simulink model "Crazyflie_Sim_CrazyDreive"  (R2026b)
settings: Solver=ode15s  StopTime=20  RelTol=1e-5
InitFcn:
  | Crazyflie_Param
values from neighbouring files (symbols this model uses):
  g = 9.80665    [Crazyflie_Param.m]
  invMix = inv(Mix)    [Crazyflie_Param.m]
  Ix_drone = 2.934e-5    (= 2.934e-05)    [Crazyflie_Param.m]
  Iy_drone = 4.981e-5    (= 4.981e-05)    [Crazyflie_Param.m]
  Iz_drone = 7.646e-5    (= 7.646e-05)    [Crazyflie_Param.m]
  J = 1/12*m*(0.051^2+0.005^2)    (= 7.878e-08)    [Crazyflie_Param.m]
  K = lqr(A, B_v, Q, R)    [Crazyflie_Param.m]
  kq = 0.006    [Crazyflie_Param.m]
  l1 = 4.445    [Crazyflie_Param.m]
  m = 0.00036    [Crazyflie_Param.m]
  m_drone = 0.04316    [Crazyflie_Param.m]
  T_e = m_tot*g/4    (= 0.1093441475)    [Crazyflie_Param.m]
undefined symbols (not defined in the file or in its folder): sigbuilder_block, X, Y, Z
libraries: sm_lib x57, nesl_utility x21, slpidlib x19, fl_lib x9
(part 1 of 4)
settings Model: Creator=BKIM  LastModifiedBy=lapsi
settings DataIOCC: ReturnWorkspaceOutputs=off
settings DebuggingCC: ArithmeticOperatorsInVariantConditions=warning
settings SFSimCC: CustomCodeUndefinedFunction=UseInterfaceOnly  SimUseLocalCustomCode=off
settings RTWCC: RTWUseLocalCustomCode=off
settings CodeAppCC: StateflowObjectComments=on
settings SimscapeCC: SimscapeNormalizeSystem=off  SimscapeUseEnergyAccounting=off
settings DiagnosticsConfigSet: SimMechanicsRigidlyBoundBlock=warning

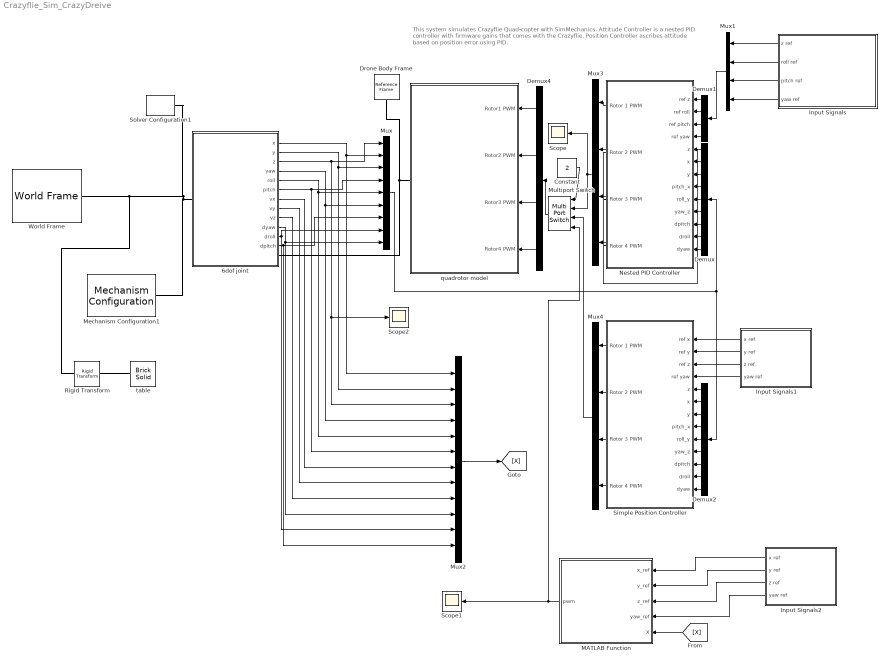
== system Crazyflie_Sim_CrazyDreive ==
  note: This system simulates Crazyflie Quad-copter with SimMechanics.
      | Attitude Controller is a nested PID controller with firmware gains that comes with the Crazyflie.
      | Position Controller ascribes attitude based on position error using PID.
  6dof joint : Subsystem
  Constant : Constant  Value=2
  Demux : Demux  Outputs=9
  Demux1 : Demux
  Demux2 : Demux  Outputs=9
  Demux4 : Demux
  Drone Body Frame : sm_lib/Frames and Transforms/Reference Frame
  Input Signals : Subsystem  Tag=STV Subsys  LoadFcn=sigbuilder_block('load');  StartFcn=sigbuilder_block('start');  StopFcn=sigbuilder_block('stop');  ClipboardFcn=sigbuilder_block('clipboard');  mask(Sigbuilder block){tuvar=[0:10]}
      mask help: Simulink:masks:SigbuilderBlock_MD
      mask init:
      | if ~strcmp(get_param(bdroot(gcbh),'SimulationStatus'),'stopped') tuvar = sigbuilder_block('maskInit'); end
      settings: CopyFcn=sigbuilder_block('copy');  DeleteFcn=sigbuilder_block('delete');  ModelCloseFcn=sigbuilder_block('modelClose');  PreSaveFcn=sigbuilder_block('preSave');  PauseFcn=sigbuilder_block('pause');  ContinueFcn=sigbuilder_block('continue');  NameChangeFcn=sigbuilder_block('namechange');  OpenFcn=sigbuilder_block('open',[6 0 1428 756 ]);  CloseFcn=sigbuilder_block('close');
      mask Display: plot(0, 0, 100, 100,[2, 2, 32, 32, 2], [68, 8, 8, 68, 68],[32, 2], [38, 38], [32, 19, 2],[53, 60, 44], [32, 17, 17, 2],[16, 16, 31, 31]);txt = getActiveGroup(gcbh);text(2, 100, txt,'verticalAlignment', 'top');
  Input Signals1 : Subsystem  Tag=STV Subsys  LoadFcn=sigbuilder_block('load');  StartFcn=sigbuilder_block('start');  StopFcn=sigbuilder_block('stop');  ClipboardFcn=sigbuilder_block('clipboard');  mask(Sigbuilder block){tuvar=[0:10]}
      mask help: Simulink:masks:SigbuilderBlock_MD
      mask init:
      | if ~strcmp(get_param(bdroot(gcbh),'SimulationStatus'),'stopped') tuvar = sigbuilder_block('maskInit'); end
      settings: CopyFcn=sigbuilder_block('copy');  DeleteFcn=sigbuilder_block('delete');  ModelCloseFcn=sigbuilder_block('modelClose');  PreSaveFcn=sigbuilder_block('preSave');  PauseFcn=sigbuilder_block('pause');  ContinueFcn=sigbuilder_block('continue');  NameChangeFcn=sigbuilder_block('namechange');  OpenFcn=sigbuilder_block('open',[441.75 141 756 505.5 ]);  CloseFcn=sigbuilder_block('close');
      mask Display: plot(0, 0, 100, 100,[2, 2, 32, 32, 2], [68, 8, 8, 68, 68],[32, 2], [38, 38], [32, 19, 2],[53, 60, 44], [32, 17, 17, 2],[16, 16, 31, 31]);txt = getActiveGroup(gcbh);text(2, 100, txt,'verticalAlignment', 'top');
  Input Signals2 : Subsystem  Tag=STV Subsys  LoadFcn=sigbuilder_block('load');  StartFcn=sigbuilder_block('start');  StopFcn=sigbuilder_block('stop');  ClipboardFcn=sigbuilder_block('clipboard');  mask(Sigbuilder block){tuvar=[0:10]}
      mask help: Simulink:masks:SigbuilderBlock_MD
      mask init:
      | if ~strcmp(get_param(bdroot(gcbh),'SimulationStatus'),'stopped') tuvar = sigbuilder_block('maskInit'); end
      settings: CopyFcn=sigbuilder_block('copy');  DeleteFcn=sigbuilder_block('delete');  ModelCloseFcn=sigbuilder_block('modelClose');  PreSaveFcn=sigbuilder_block('preSave');  PauseFcn=sigbuilder_block('pause');  ContinueFcn=sigbuilder_block('continue');  NameChangeFcn=sigbuilder_block('namechange');  OpenFcn=sigbuilder_block('open',[441.75 141 756 505.5 ]);  CloseFcn=sigbuilder_block('close');
      mask Display: plot(0, 0, 100, 100,[2, 2, 32, 32, 2], [68, 8, 8, 68, 68],[32, 2], [38, 38], [32, 19, 2],[53, 60, 44], [32, 17, 17, 2],[16, 16, 31, 31]);txt = getActiveGroup(gcbh);text(2, 100, txt,'verticalAlignment', 'top');
  MATLAB Function : MATLAB Function  TreatAsAtomicUnit=on
  Mechanism Configuration1 : sm_lib/Utilities/Mechanism Configuration  UniformGravity=Constant  GravityVector=[0 0 -g]  GravityVectorUnits=m/s^2  LinearizationDelta=0.001  JointModeTransitionNonlinearIterations=2
  Multiport Switch : MultiPortSwitch  SaturateOnIntegerOverflow=off  InputSameDT=off
  Mux : Mux  Inputs=9
  Mux1 : Mux
  Mux2 : Mux  Inputs=12
  Mux3 : Mux
  Mux4 : Mux
  Nested PID Controller : Subsystem
  Rigid Transform : sm_lib/Frames and Transforms/Rigid Transform  RotationMethod=None  FollAlignAxisA=+X  BaseAlignAxisA=+Y  FollAlignAxisB=+Y  BaseAlignAxisB=+Z  RotationStandardAxis=+Z  RotationAngle=0  RotationAngleUnits=deg  RotationArbitraryAxis=[0 0 1]  RotationSequenceAxes=FollowerAxes  RotationSequence=XYX  RotationSequenceAngles=[0 0 0]  RotationSequenceAnglesUnits=deg  RotationMatrix=[1 0 0;0 1 0;0 0 1]  Quaternion=[1 0 0 0]  TranslationMethod=Cartesian  TranslationCartesianOffset=[2 0 0.95]  TranslationCartesianOffsetUnits=m  TranslationStandardAxis=+Z  TranslationStandardOffset=0  TranslationStandardOffsetUnits=m  TranslationROffset=0  TranslationROffsetUnits=m  TranslationThetaOffset=0  TranslationThetaOffsetUnits=deg  TranslationZOffset=0  TranslationZOffsetUnits=m
  Scope : Scope
  Scope1 : Scope
      settings: ActiveDisplayYMinimum=27214.451130136935  ActiveDisplayYMaximum=69792.838763318112  DataLoggingVariableName=ScopeData4
  Scope2 : Scope
      settings: ActiveDisplayYMinimum=-0.25000006411505821  ActiveDisplayYMaximum=2.2500005770355243  DataLoggingVariableName=ScopeData5
  Simple Position Controller : Subsystem
  Solver Configuration1 : nesl_utility/Solver Configuration  PhysicalDomain=network_engine_domain  SubClassName=solver  LeftPortType=input  RightPortType=generic  Tones=[]  Harmonics=[]  SimulateNoise=off  Profile=off  UseLocalSampling=off  EnableSwitchedLinearOptims=on  FrequencyDomain=off  UseCCode=off  RelTol=0.001  AbsTol=1e-06  MinStep=1e-09  ToWorkspace=off  RevertToSquareIcSolve=off  NumHomotopyIterations=100  PhasorMode=off  PhasorModeNumHarmonics=1  ConsistencySolver=NEWTON_FTOL  CanonicalOrdering=UNORDERED  OptimizeIntermediates=UNOPTIMIZED  MulticoreSolverChoice=BACKWARD_EULER  IndexReductionMethod=DerivativeReplacement  DoDC=off  ResidualTolerance=1e-09  ConsistencyTolSource=GLOBAL  ConsistencyAbsTol=0.001  ConsistencyRelTol=0.001  ConsistencyTolFactor=0.001  UseLocalSolver=off  LocalSolverChoice=NE_BACKWARD_EULER_ADVANCER  ResolveIndetEquations=on  FunctionEvalNumThread=1  LocalSolverSampleTime=0.001  DoFixedCost=off  MaxNonlinIter=3  MaxModeIter=2  ComputeImpulses=off  ImpulseIterations=2  LinearAlgebra=Sparse  LinearAlgebraNumThread=0  EquationFormulation=NE_TIME_EF  DelaysMemoryBudget=1024  AutomaticFiltering=on  FilteringTimeConstant=0.001  PartitionStorageMethod=AS_NEEDED  PartitionMemoryBudget=1024  PartitionMethod=FAST  MultibodyUseLocalSolver=off  MultibodyLocalSolverChoice=ODE1  MultibodyLocalSolverSampleTime=0.001
  World Frame : sm_lib/Frames and Transforms/World Frame
  quadrotor model : Subsystem
  table : sm_lib/Body Elements/Brick Solid  BrickDimensions=[2.5 0.6 0.1]  BrickDimensionsUnits=m  ExportEntireGeometry=off  InertiaType=CalculateFromGeometry  BasedOnType=Density  Density=1000  DensityUnits=kg/m^3  Mass=1  MassUnits=kg  CenterOfMass=[0 0 0]  CenterOfMassUnits=m  MomentsOfInertia=[1 1 1]  MomentsOfInertiaUnits=kg*m^2  ProductsOfInertia=[0 0 0]  ProductsOfInertiaUnits=kg*m^2  GraphicType=FromGeometry  MarkerShape=Sphere  MarkerSize=10  GraphicVisPropType=AdvancedVisualProperties  GraphicDiffuseColor=[0.5 0.5 0.5]  GraphicOpacity=1  GraphicSpecularColor=[0.5 0.5 0.5 1.0]  GraphicAmbientColor=[0.15 0.15 0.15 1.0]  GraphicEmissiveColor=[0.0 0.0 0.0 1.0]  GraphicShininess=75  DoExposeReferenceFrame=on  SerializedFrames=<Frames/>
  wires:
  6dof joint/3(z) -> Mux2/3, Scope2/1, Mux/1
  6dof joint/1(x) -> Mux2/1, Mux/2
  6dof joint/2(y) -> Mux2/2, Mux/3
  6dof joint/6(pitch) -> Mux2/6, Mux/4
  6dof joint/5(roll) -> Mux2/5, Mux/5
  6dof joint/4(yaw) -> Mux2/4, Mux/6
  6dof joint/12(dpitch) -> Mux2/12, Mux/7
  6dof joint/11(droll) -> Mux2/11, Mux/8
  6dof joint/10(dyaw) -> Mux2/10, Mux/9
  Demux/1 -> Nested PID Controller/5(z)
  Demux/2 -> Nested PID Controller/6(x)
  Demux/3 -> Nested PID Controller/7(y)
  Demux/4 -> Nested PID Controller/8(pitch_x)
  Demux/5 -> Nested PID Controller/9(roll_y)
  Demux/6 -> Nested PID Controller/10(yaw_z)
  Demux/7 -> Nested PID Controller/11(dpitch)
  Demux/8 -> Nested PID Controller/12(droll)
  Demux/9 -> Nested PID Controller/13(dyaw)
  Input Signals/1(z ref) -> Mux1/1
  Input Signals/2(roll ref) -> Mux1/2
  Input Signals/3(pitch ref) -> Mux1/3
  Input Signals/4(yaw ref) -> Mux1/4
  Demux1/2 -> Nested PID Controller/2(ref roll)
  Demux1/1 -> Nested PID Controller/1(ref z)
  Demux1/3 -> Nested PID Controller/3(ref pitch)
  Demux1/4 -> Nested PID Controller/4(ref yaw)
  Mux1/1 -> Demux1/1
  Demux4/1 -> quadrotor model/1(Rotor1 PWM)
  Demux4/2 -> quadrotor model/2(Rotor2 PWM)
  Demux4/3 -> quadrotor model/3(Rotor3 PWM)
  Demux4/4 -> quadrotor model/4(Rotor4 PWM)
  Nested PID Controller/1(Rotor 1 PWM) -> Mux3/1
  Nested PID Controller/2(Rotor 2 PWM) -> Mux3/2
  Nested PID Controller/3(Rotor 3 PWM) -> Mux3/3
  Nested PID Controller/4(Rotor 4 PWM) -> Mux3/4
  Demux2/3 -> Simple Position Controller/7(y)
  Demux2/7 -> Simple Position Controller/11(dpitch)
  Simple Position Controller/4(Rotor 4 PWM) -> Mux4/4
  Simple Position Controller/3(Rotor 3 PWM) -> Mux4/3
  Demux2/9 -> Simple Position Controller/13(dyaw)
  Simple Position Controller/2(Rotor 2 PWM) -> Mux4/2
  Demux2/4 -> Simple Position Controller/8(pitch_x)
  Demux2/2 -> Simple Position Controller/6(x)
  Mux/1 -> Demux2/1, Demux/1
  Demux2/6 -> Simple Position Controller/10(yaw_z)
  Demux2/8 -> Simple Position Controller/12(droll)
  Demux2/1 -> Simple Position Controller/5(z)
  Demux2/5 -> Simple Position Controller/9(roll_y)
  Simple Position Controller/1(Rotor 1 PWM) -> Mux4/1
  Multiport Switch/1 -> Demux4/1
  Input Signals1/3(z ref) -> Simple Position Controller/3(ref z)
  Input Signals1/2(y ref) -> Simple Position Controller/2(ref y)
  Input Signals1/1(x ref) -> Simple Position Controller/1(ref x)
  Input Signals1/4(yaw ref) -> Simple Position Controller/4(ref yaw)
  Mux2/1 -> [X]
  [X] -> MATLAB Function/5(X)
  Mux3/1 -> Multiport Switch/2, Scope/1
  Mux4/1 -> Multiport Switch/3
  MATLAB Function/1(pwm) -> Scope1/1, Multiport Switch/4
  6dof joint/7(vx) -> Mux2/7
  6dof joint/8(vy) -> Mux2/8
  6dof joint/9(vz) -> Mux2/9
  Constant/1 -> Multiport Switch/1
  Input Signals2/1(x ref) -> MATLAB Function/1(x_ref)
  Input Signals2/2(y ref) -> MATLAB Function/2(y_ref)
  Input Signals2/3(z ref) -> MATLAB Function/3(z_ref)
  Input Signals2/4(yaw ref) -> MATLAB Function/4(yaw_ref)
  connections:
  6dof joint/LConn1 -- Solver Configuration1/RConn1 -- Rigid Transform/LConn1 -- World Frame/RConn1 -- Mechanism Configuration1/RConn1
  Drone Body Frame/RConn1 -- 6dof joint/RConn1 -- quadrotor model/RConn1
  Rigid Transform/RConn1 -- table/RConn1

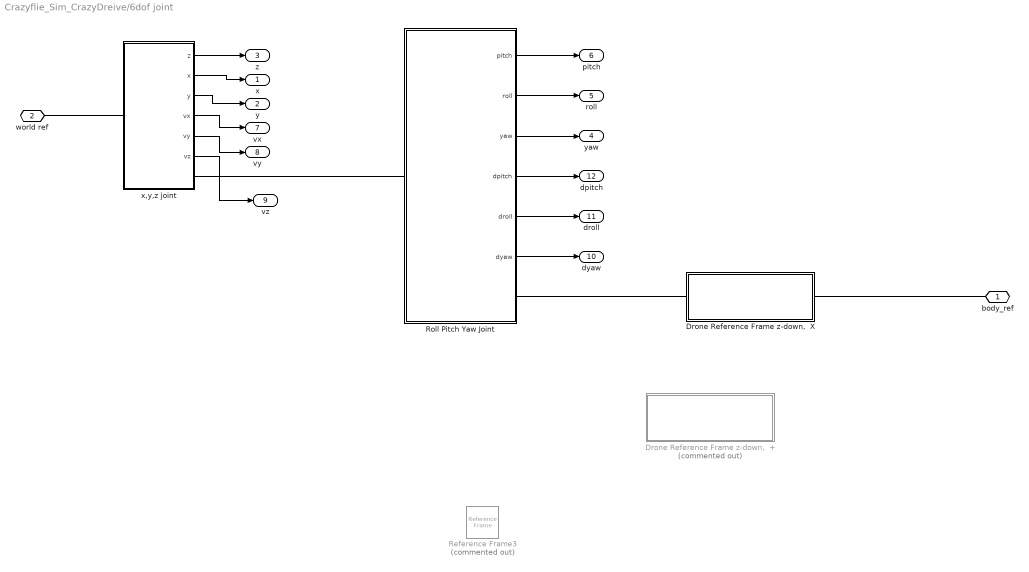
== system Crazyflie_Sim_CrazyDreive/6dof joint ==
  "Drone Reference Frame z-down,  +" : Subsystem  Commented=on
  "Drone Reference Frame z-down,  X " : Subsystem
  Reference Frame3 : sm_lib/Frames and Transforms/Reference Frame  Commented=on
  Roll Pitch Yaw Joint : Subsystem
  x,y,z joint : Subsystem
  body_ref : PMIOPort  Side=Right
  world ref : PMIOPort  Port=2  Side=Left
  x : Outport
  y : Outport  Port=2
  z : Outport  Port=3
  yaw : Outport  Port=4
  roll : Outport  Port=5
  pitch : Outport  Port=6
  vx : Outport  Port=7
  vy : Outport  Port=8
  vz : Outport  Port=9
  dyaw : Outport  Port=10
  droll : Outport  Port=11
  dpitch : Outport  Port=12
  wires:
  x,y,z joint/1(z) -> z/1
  x,y,z joint/2(x) -> x/1
  x,y,z joint/3(y) -> y/1
  Roll Pitch Yaw Joint/1(pitch) -> pitch/1
  Roll Pitch Yaw Joint/2(roll) -> roll/1
  Roll Pitch Yaw Joint/3(yaw) -> yaw/1
  Roll Pitch Yaw Joint/4(dpitch) -> dpitch/1
  Roll Pitch Yaw Joint/5(droll) -> droll/1
  Roll Pitch Yaw Joint/6(dyaw) -> dyaw/1
  x,y,z joint/4(vx) -> vx/1
  x,y,z joint/5(vy) -> vy/1
  x,y,z joint/6(vz) -> vz/1
  connections:
  world ref/RConn1 -- x,y,z joint/LConn1
  x,y,z joint/RConn1 -- Roll Pitch Yaw Joint/LConn1
  "Drone Reference Frame z-down,  X "/RConn1 -- body_ref/RConn1
  "Drone Reference Frame z-down,  X "/LConn1 -- Roll Pitch Yaw Joint/RConn1

== system Crazyflie_Sim_CrazyDreive/Input Signals ==
  Demux : Demux  Tag=STV Demux
      settings: DisplayOption=none
  FromWs : FromWorkspace  Tag=STV FromWs  VariableName=tuvar
      SigBuilderData=|
      | common.afterFinalStr = 'Extrapolate'
      | common.sampleTime = 0
      | dataSet.timeRange = [0 30]
      | dataSet.name = 'Group 1'
      | sbobj.Groups.Name = 'Group 1'
      | sbobj.Groups.Signals(1).Name = 'z ref'
      | sbobj.Groups.Signals(1).XData = [0 5 30]
      | sbobj.Groups.Signals(1).YData = [0 0.99 0.99]
      | sbobj.Groups.Signals(2).Name = 'roll ref'
      | sbobj.Groups.Signals(2).XData = [0 6 6.5 7 7.5 8 8.5 11 11.5 12 12.5 13 30]
      | sbobj.Groups.Signals(2).YData = [0 0 0.35 0.35 -0.35 -0.35 0 0 0.1 0 -0.1 0 0]
      | sbobj.Groups.Signals(3).Name = 'pitch ref'
      | sbobj.Groups.Signals(3).XData = [0 9 9.5 10 10.5 11 11.5 12 12.5 25 30]
      | sbobj.Groups.Signals(3).YData = [0 0 -0.35 0.35 0 0 -0.1 0.1 0 0 0]
      | sbobj.Groups.Signals(4).Name = 'yaw ref'
      | sbobj.Groups.Signals(4).XData = [0 5 6 15 15 19 19 23 24 25 26 30]
      | sbobj.Groups.Signals(4).YData = [0 0 0 0 0.52 0.52 0 0 0 0 0 0]
      | sbobj.Groups.TimeRange = [0 30]
  z ref : Outport  Tag=STV Outport
  roll ref : Outport  Tag=STV Outport  Port=2
  pitch ref : Outport  Tag=STV Outport  Port=3
  yaw ref : Outport  Tag=STV Outport  Port=4
  wires:
  FromWs/1 -> Demux/1
  Demux/1 -> z ref/1
  Demux/2 -> roll ref/1
  Demux/3 -> pitch ref/1
  Demux/4 -> yaw ref/1

== system Crazyflie_Sim_CrazyDreive/Input Signals1 ==
  Demux : Demux  Tag=STV Demux
      settings: DisplayOption=none
  FromWs : FromWorkspace  Tag=STV FromWs  VariableName=tuvar
      SigBuilderData=|
      | common.afterFinalStr = 'Extrapolate'
      | common.sampleTime = 0
      | dataSet.timeRange = [0 25]
      | dataSet.name = 'Group 1'
      | sbobj.Groups.Name = 'Group 1'
      | sbobj.Groups.Signals(1).Name = 'x ref'
      | sbobj.Groups.Signals(1).XData = [0 5 5.5 6 6.5 7 7.5 8 8.5 9 9.5 10 10.5 11 11.5 12 12.5 13 25]
      | sbobj.Groups.Signals(1).YData = [0 0 0 0 0 0 0 0 0 0 0 0 0 0 0 0 0 1 1]
      | sbobj.Groups.Signals(2).Name = 'y ref'
      | sbobj.Groups.Signals(2).XData = [0 5 5.5 6 6.5 7 7.5 8 8.5 9 9.5 10 10.5 11 11.5 12 12.5 13 25]
      | sbobj.Groups.Signals(2).YData = [0 0 0 0 0 0 0 0 0 0 0 0 0 0 0 0 0 0 0]
      | sbobj.Groups.Signals(3).Name = 'z ref'
      | sbobj.Groups.Signals(3).XData = [0 5 13 18 25]
      | sbobj.Groups.Signals(3).YData = [0 2 2 1.05 1.05]
      | sbobj.Groups.Signals(4).Name = 'yaw ref'
      | sbobj.Groups.Signals(4).XData = [0 23 24 25]
      | sbobj.Groups.Signals(4).YData = [0 0 0 0]
      | sbobj.Groups.TimeRange = [0 25]
  x ref : Outport  Tag=STV Outport
  y ref : Outport  Tag=STV Outport  Port=2
  z ref : Outport  Tag=STV Outport  Port=3
  yaw ref : Outport  Tag=STV Outport  Port=4
  wires:
  FromWs/1 -> Demux/1
  Demux/1 -> x ref/1
  Demux/2 -> y ref/1
  Demux/3 -> z ref/1
  Demux/4 -> yaw ref/1

== system Crazyflie_Sim_CrazyDreive/Input Signals2 ==
  Demux : Demux  Tag=STV Demux
      settings: DisplayOption=none
  FromWs : FromWorkspace  Tag=STV FromWs  VariableName=tuvar
      SigBuilderData=|
      | common.afterFinalStr = 'Extrapolate'
      | common.sampleTime = 0
      | dataSet.timeRange = [0 25]
      | dataSet.name = 'Group 1'
      | sbobj.Groups.Name = 'Group 1'
      | sbobj.Groups.Signals(1).Name = 'x ref'
      | sbobj.Groups.Signals(1).XData = [0 5 5.5 6 6.5 7 7.5 8 8.5 9 9.5 10 10.5 11 11.5 12 12.5 13 25]
      | sbobj.Groups.Signals(1).YData = [0 0 0 0 0 0 0 0 0 0 0 0 0 0 0 0 0 1 1]
      | sbobj.Groups.Signals(2).Name = 'y ref'
      | sbobj.Groups.Signals(2).XData = [0 5 5.5 6 6.5 7 7.5 8 8.5 9 9.5 10 10.5 11 11.5 12 12.5 13 25]
      | sbobj.Groups.Signals(2).YData = [0 0 0 0 0 0 0 0 0 0 0 0 0 0 0 0 0 0 0]
      | sbobj.Groups.Signals(3).Name = 'z ref'
      | sbobj.Groups.Signals(3).XData = [0 5 13 18 25]
      | sbobj.Groups.Signals(3).YData = [0 2 2 1.05 1.05]
      | sbobj.Groups.Signals(4).Name = 'yaw ref'
      | sbobj.Groups.Signals(4).XData = [0 23 24 25]
      | sbobj.Groups.Signals(4).YData = [0 0 0 0]
      | sbobj.Groups.TimeRange = [0 25]
  x ref : Outport  Tag=STV Outport
  y ref : Outport  Tag=STV Outport  Port=2
  z ref : Outport  Tag=STV Outport  Port=3
  yaw ref : Outport  Tag=STV Outport  Port=4
  wires:
  Demux/4 -> yaw ref/1
  Demux/3 -> z ref/1
  Demux/2 -> y ref/1
  Demux/1 -> x ref/1
  FromWs/1 -> Demux/1

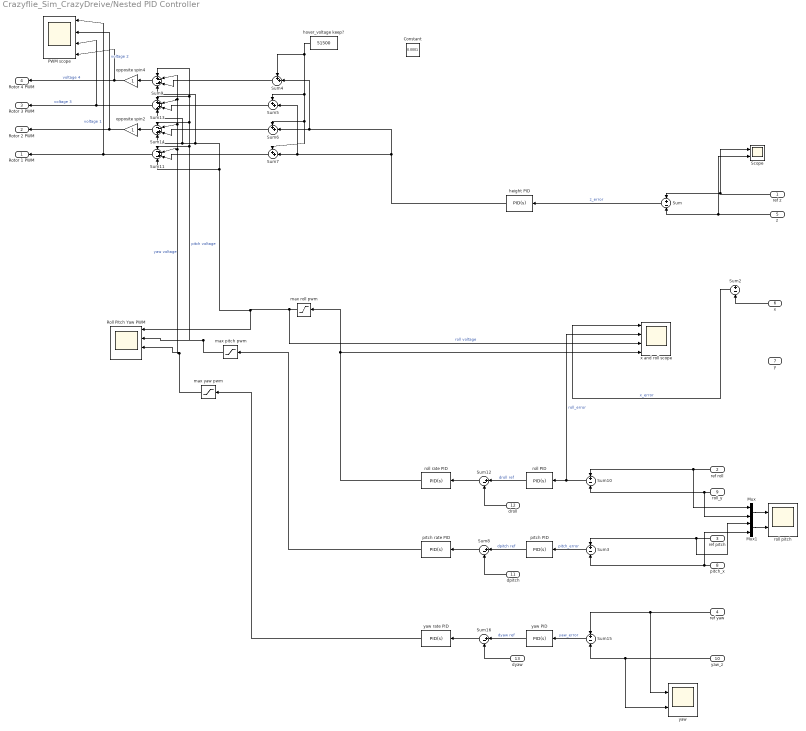
== system Crazyflie_Sim_CrazyDreive/Nested PID Controller ==
  ref z : Inport
  ref roll : Inport  Port=2
  ref pitch : Inport  Port=3
  ref yaw : Inport  Port=4
  z : Inport  Port=5
  x : Inport  Port=6
  y : Inport  Port=7
  pitch_x : Inport  Port=8
  roll_y : Inport  Port=9
  yaw_z : Inport  Port=10
  dpitch : Inport  Port=11
  droll : Inport  Port=12
  dyaw : Inport  Port=13
  Constant : Constant  Value=0.0001
  Mux : Mux  Inputs=2
  Mux1 : Mux  Inputs=2
  PWM scope : Scope  NumInputPorts=4
      settings: ActiveDisplayYMinimum=30000  ActiveDisplayYMaximum=50000
  Roll Pitch Yaw PWM : Scope  NumInputPorts=4
      settings: ActiveDisplayYMinimum=-81918.75  ActiveDisplayYMaximum=81918.75
  Scope : Scope  NumInputPorts=2
      settings: ActiveDisplayYMinimum=-0.12883916669712672  ActiveDisplayYMaximum=1.1595525002741407  DataLoggingVariableName=ScopeData2
  Sum{,2..3,10,15} (5 alike) : Sum  Inputs=+-
  Sum11 : Sum  Inputs=-++-
  Sum12 : Sum  Inputs=|+-
  Sum13 : Sum  Inputs=++++
  Sum14 : Sum  Inputs=--++
  Sum16 : Sum  Inputs=|+-
  Sum{4..7} (4 alike) : Sum  Inputs=++|
  Sum8 : Sum  Inputs=|+-
  Sum9 : Sum  Inputs=+-+-
  height PID : slpidlib/PID Controller  Controller=PID  Form=Parallel  TimeDomain=Continuous-time  UseExternalTs=off  SampleTime=-1  IntegratorMethod=Forward Euler  FilterMethod=Forward Euler  ControllerParametersSource=internal  P=20000  I=0  UseKiTs=off  D=10000  UseExternalDerivativeSource=off  N=100  UseFilter=on  TunerSelectOption=Transfer Function Based (PID Tuner App)  InitialConditionSource=internal  InitialConditionForIntegrator=0  InitialConditionForFilter=0  DifferentiatorICPrevScaledInput=0  ExternalReset=none  TrackingMode=off  Kt=1  LimitOutput=off  SatLimitsSource=internal  UpperSaturationLimit=inf  LowerSaturationLimit=-inf  LinearizeAsGain=on  AntiWindupMode=none  Kb=1  LimitIntegrator=off  UpperIntegratorSaturationLimit=inf  LowerIntegratorSaturationLimit=-inf  POutMin=[]  POutMax=[]  IOutMin=[]  IOutMax=[]  DOutMin=[]  DOutMax=[]  NOutMin=[]  NOutMax=[]  SumOutMin=[]  SumOutMax=[]  SaturationOutMin=[]  SaturationOutMax=[]  PParamMin=[]  PParamMax=[]  IParamMin=[]  IParamMax=[]  DParamMin=[]  DParamMax=[]  NParamMin=[]  NParamMax=[]  KbParamMin=[]  KbParamMax=[]  KtParamMin=[]  KtParamMax=[]  KbOutMin=[]  KbOutMax=[]  KtOutMin=[]  KtOutMax=[]  IntegratorOutMin=[]  IntegratorOutMax=[]  FilterOutMin=[]  FilterOutMax=[]  SumI1OutMin=[]  SumI1OutMax=[]  SumI2OutMin=[]  SumI2OutMax=[]  SumI3OutMin=[]  SumI3OutMax=[]  SumI4OutMin=[]  SumI4OutMax=[]  SumDOutMin=[]  SumDOutMax=[]  DifferentiatorOutMin=[]  DifferentiatorOutMax=[]  FilterDiffOutCoefMin=[]  FilterDiffOutCoefMax=[]  ReciprocalOutMin=[]  ReciprocalOutMax=[]  SumDenOutMin=[]  SumDenOutMax=[]  SumNumOutMin=[]  SumNumOutMax=[]  DivideOutMin=[]  DivideOutMax=[]  UdiffTsProdOutMin=[]  UdiffTsProdOutMax=[]  NTsProdOutMin=[]  NTsProdOutMax=[]  UintegralTsProdOutMin=[]  UintegralTsProdOutMax=[]  UngainTsProdOutMin=[]  UngainTsProdOutMax=[]  ClampingZeroOutDataTypeStr=Inherit: Inherit via back propagation  ClampingZeroOutMin=[]  ClampingZeroOutMax=[]  FilterDenConstantOutDataTypeStr=Inherit: Inherit via back propagation  FilterDenConstantOutMin=[]  FilterDenConstantOutMax=[]  PCopyOutDataTypeStr=Inherit: Inherit via back propagation  PCopyOutMin=[]  PCopyOutMax=[]  NCopyOutDataTypeStr=Inherit: Inherit via back propagation  NCopyOutMin=[]  NCopyOutMax=[]  IntegratorContinuousStateAttributes=''  IntegratorStateMustResolveToSignalObject=off  IntegratorRTWStateStorageClass=Auto  FilterContinuousStateAttributes=''  FilterStateMustResolveToSignalObject=off  FilterRTWStateStorageClass=Auto  ParallelPVariant=InternalParameters  IdealPVariant=Disabled  IVariant=InternalParameters  DVariant=InternalParameters  IntegratorVariant=Continuous  SatVariant=Disabled  AWVariant=Passthrough  PCopyVariant=Disabled  TRVariant=Disabled  FdbkBlocksVariant=Forward  IdealPFdbkVariant=Disabled  SatFdbkVariant=Disabled  DerivativeFilterVariant=ContFilter  NVariant=InternalParameters  NCopyVariant=Disabled  FilterICVariant=InternalICsFilter  IntegratorICVariant=InternalICs  ExternalResetVariant=Disabled  TRSumVariant=Passthrough  SumFdbkVariant=Disabled  SumVariant=Sum_PID  TsampFilterVariant=InternalTs  TsampNgainVariant=Passthrough  TsampIntegralVariant=Disabled_SignalSpec  ExternalSaturationOutDataTypeStr=Inherit: Same as second input  DerivativeSourceVariant=ErrorSignal  PreIntVariant=InternalPreInt
  hover_voltage keep? : Constant  Value=51500
  max pitch pwm : Saturate  UpperLimit=65535  LowerLimit=-65535  ZeroCross=off
  max roll pwm : Saturate  UpperLimit=65535  LowerLimit=-65535  ZeroCross=off
  max yaw pwm : Saturate  UpperLimit=65535  LowerLimit=-65535  ZeroCross=off
  opposite spin2 : Gain
  opposite spin4 : Gain
  pitch PID : slpidlib/PID Controller  Controller=PID  Form=Parallel  TimeDomain=Continuous-time  UseExternalTs=off  SampleTime=-1  IntegratorMethod=Forward Euler  FilterMethod=Forward Euler  ControllerParametersSource=internal  P=6  I=3  UseKiTs=off  D=0  UseExternalDerivativeSource=off  N=100  UseFilter=on  TunerSelectOption=Transfer Function Based (PID Tuner App)  InitialConditionSource=internal  InitialConditionForIntegrator=0  InitialConditionForFilter=0  DifferentiatorICPrevScaledInput=0  ExternalReset=none  TrackingMode=off  Kt=1  LimitOutput=off  SatLimitsSource=internal  UpperSaturationLimit=inf  LowerSaturationLimit=-inf  LinearizeAsGain=on  AntiWindupMode=none  Kb=1  LimitIntegrator=off  UpperIntegratorSaturationLimit=inf  LowerIntegratorSaturationLimit=-inf  POutMin=[]  POutMax=[]  IOutMin=[]  IOutMax=[]  DOutMin=[]  DOutMax=[]  NOutMin=[]  NOutMax=[]  SumOutMin=[]  SumOutMax=[]  SaturationOutMin=[]  SaturationOutMax=[]  PParamMin=[]  PParamMax=[]  IParamMin=[]  IParamMax=[]  DParamMin=[]  DParamMax=[]  NParamMin=[]  NParamMax=[]  KbParamMin=[]  KbParamMax=[]  KtParamMin=[]  KtParamMax=[]  KbOutMin=[]  KbOutMax=[]  KtOutMin=[]  KtOutMax=[]  IntegratorOutMin=[]  IntegratorOutMax=[]  FilterOutMin=[]  FilterOutMax=[]  SumI1OutMin=[]  SumI1OutMax=[]  SumI2OutMin=[]  SumI2OutMax=[]  SumI3OutMin=[]  SumI3OutMax=[]  SumI4OutMin=[]  SumI4OutMax=[]  SumDOutMin=[]  SumDOutMax=[]  DifferentiatorOutMin=[]  DifferentiatorOutMax=[]  FilterDiffOutCoefMin=[]  FilterDiffOutCoefMax=[]  ReciprocalOutMin=[]  ReciprocalOutMax=[]  SumDenOutMin=[]  SumDenOutMax=[]  SumNumOutMin=[]  SumNumOutMax=[]  DivideOutMin=[]  DivideOutMax=[]  UdiffTsProdOutMin=[]  UdiffTsProdOutMax=[]  NTsProdOutMin=[]  NTsProdOutMax=[]  UintegralTsProdOutMin=[]  UintegralTsProdOutMax=[]  UngainTsProdOutMin=[]  UngainTsProdOutMax=[]  ClampingZeroOutDataTypeStr=Inherit: Inherit via back propagation  ClampingZeroOutMin=[]  ClampingZeroOutMax=[]  FilterDenConstantOutDataTypeStr=Inherit: Inherit via back propagation  FilterDenConstantOutMin=[]  FilterDenConstantOutMax=[]  PCopyOutDataTypeStr=Inherit: Inherit via back propagation  PCopyOutMin=[]  PCopyOutMax=[]  NCopyOutDataTypeStr=Inherit: Inherit via back propagation  NCopyOutMin=[]  NCopyOutMax=[]  IntegratorContinuousStateAttributes=''  IntegratorStateMustResolveToSignalObject=off  IntegratorRTWStateStorageClass=Auto  FilterContinuousStateAttributes=''  FilterStateMustResolveToSignalObject=off  FilterRTWStateStorageClass=Auto  ParallelPVariant=InternalParameters  IdealPVariant=Disabled  IVariant=InternalParameters  DVariant=InternalParameters  IntegratorVariant=Continuous  SatVariant=Disabled  AWVariant=Passthrough  PCopyVariant=Disabled  TRVariant=Disabled  FdbkBlocksVariant=Forward  IdealPFdbkVariant=Disabled  SatFdbkVariant=Disabled  DerivativeFilterVariant=ContFilter  NVariant=InternalParameters  NCopyVariant=Disabled  FilterICVariant=InternalICsFilter  IntegratorICVariant=InternalICs  ExternalResetVariant=Disabled  TRSumVariant=Passthrough  SumFdbkVariant=Disabled  SumVariant=Sum_PID  TsampFilterVariant=InternalTs  TsampNgainVariant=Passthrough  TsampIntegralVariant=Disabled_SignalSpec  ExternalSaturationOutDataTypeStr=Inherit: Same as second input  DerivativeSourceVariant=ErrorSignal  PreIntVariant=InternalPreInt
  pitch rate PID : slpidlib/PID Controller  Controller=PID  Form=Parallel  TimeDomain=Continuous-time  UseExternalTs=off  SampleTime=-1  IntegratorMethod=Forward Euler  FilterMethod=Forward Euler  ControllerParametersSource=internal  P=750  I=1500  UseKiTs=off  D=7.5  UseExternalDerivativeSource=off  N=100  UseFilter=on  TunerSelectOption=Transfer Function Based (PID Tuner App)  InitialConditionSource=internal  InitialConditionForIntegrator=0  InitialConditionForFilter=0  DifferentiatorICPrevScaledInput=0  ExternalReset=none  TrackingMode=off  Kt=1  LimitOutput=off  SatLimitsSource=internal  UpperSaturationLimit=inf  LowerSaturationLimit=-inf  LinearizeAsGain=on  AntiWindupMode=none  Kb=1  LimitIntegrator=off  UpperIntegratorSaturationLimit=inf  LowerIntegratorSaturationLimit=-inf  POutMin=[]  POutMax=[]  IOutMin=[]  IOutMax=[]  DOutMin=[]  DOutMax=[]  NOutMin=[]  NOutMax=[]  SumOutMin=[]  SumOutMax=[]  SaturationOutMin=[]  SaturationOutMax=[]  PParamMin=[]  PParamMax=[]  IParamMin=[]  IParamMax=[]  DParamMin=[]  DParamMax=[]  NParamMin=[]  NParamMax=[]  KbParamMin=[]  KbParamMax=[]  KtParamMin=[]  KtParamMax=[]  KbOutMin=[]  KbOutMax=[]  KtOutMin=[]  KtOutMax=[]  IntegratorOutMin=[]  IntegratorOutMax=[]  FilterOutMin=[]  FilterOutMax=[]  SumI1OutMin=[]  SumI1OutMax=[]  SumI2OutMin=[]  SumI2OutMax=[]  SumI3OutMin=[]  SumI3OutMax=[]  SumI4OutMin=[]  SumI4OutMax=[]  SumDOutMin=[]  SumDOutMax=[]  DifferentiatorOutMin=[]  DifferentiatorOutMax=[]  FilterDiffOutCoefMin=[]  FilterDiffOutCoefMax=[]  ReciprocalOutMin=[]  ReciprocalOutMax=[]  SumDenOutMin=[]  SumDenOutMax=[]  SumNumOutMin=[]  SumNumOutMax=[]  DivideOutMin=[]  DivideOutMax=[]  UdiffTsProdOutMin=[]  UdiffTsProdOutMax=[]  NTsProdOutMin=[]  NTsProdOutMax=[]  UintegralTsProdOutMin=[]  UintegralTsProdOutMax=[]  UngainTsProdOutMin=[]  UngainTsProdOutMax=[]  ClampingZeroOutDataTypeStr=Inherit: Inherit via back propagation  ClampingZeroOutMin=[]  ClampingZeroOutMax=[]  FilterDenConstantOutDataTypeStr=Inherit: Inherit via back propagation  FilterDenConstantOutMin=[]  FilterDenConstantOutMax=[]  PCopyOutDataTypeStr=Inherit: Inherit via back propagation  PCopyOutMin=[]  PCopyOutMax=[]  NCopyOutDataTypeStr=Inherit: Inherit via back propagation  NCopyOutMin=[]  NCopyOutMax=[]  IntegratorContinuousStateAttributes=''  IntegratorStateMustResolveToSignalObject=off  IntegratorRTWStateStorageClass=Auto  FilterContinuousStateAttributes=''  FilterStateMustResolveToSignalObject=off  FilterRTWStateStorageClass=Auto  ParallelPVariant=InternalParameters  IdealPVariant=Disabled  IVariant=InternalParameters  DVariant=InternalParameters  IntegratorVariant=Continuous  SatVariant=Disabled  AWVariant=Passthrough  PCopyVariant=Disabled  TRVariant=Disabled  FdbkBlocksVariant=Forward  IdealPFdbkVariant=Disabled  SatFdbkVariant=Disabled  DerivativeFilterVariant=ContFilter  NVariant=InternalParameters  NCopyVariant=Disabled  FilterICVariant=InternalICsFilter  IntegratorICVariant=InternalICs  ExternalResetVariant=Disabled  TRSumVariant=Passthrough  SumFdbkVariant=Disabled  SumVariant=Sum_PID  TsampFilterVariant=InternalTs  TsampNgainVariant=Passthrough  TsampIntegralVariant=Disabled_SignalSpec  ExternalSaturationOutDataTypeStr=Inherit: Same as second input  DerivativeSourceVariant=ErrorSignal  PreIntVariant=InternalPreInt
  roll PID : slpidlib/PID Controller  Controller=PID  Form=Parallel  TimeDomain=Continuous-time  UseExternalTs=off  SampleTime=-1  IntegratorMethod=Forward Euler  FilterMethod=Forward Euler  ControllerParametersSource=internal  P=6  I=3  UseKiTs=off  D=0  UseExternalDerivativeSource=off  N=100  UseFilter=on  TunerSelectOption=Transfer Function Based (PID Tuner App)  InitialConditionSource=internal  InitialConditionForIntegrator=0  InitialConditionForFilter=0  DifferentiatorICPrevScaledInput=0  ExternalReset=none  TrackingMode=off  Kt=1  LimitOutput=off  SatLimitsSource=internal  UpperSaturationLimit=inf  LowerSaturationLimit=-inf  LinearizeAsGain=on  AntiWindupMode=none  Kb=1  LimitIntegrator=off  UpperIntegratorSaturationLimit=inf  LowerIntegratorSaturationLimit=-inf  POutMin=[]  POutMax=[]  IOutMin=[]  IOutMax=[]  DOutMin=[]  DOutMax=[]  NOutMin=[]  NOutMax=[]  SumOutMin=[]  SumOutMax=[]  SaturationOutMin=[]  SaturationOutMax=[]  PParamMin=[]  PParamMax=[]  IParamMin=[]  IParamMax=[]  DParamMin=[]  DParamMax=[]  NParamMin=[]  NParamMax=[]  KbParamMin=[]  KbParamMax=[]  KtParamMin=[]  KtParamMax=[]  KbOutMin=[]  KbOutMax=[]  KtOutMin=[]  KtOutMax=[]  IntegratorOutMin=[]  IntegratorOutMax=[]  FilterOutMin=[]  FilterOutMax=[]  SumI1OutMin=[]  SumI1OutMax=[]  SumI2OutMin=[]  SumI2OutMax=[]  SumI3OutMin=[]  SumI3OutMax=[]  SumI4OutMin=[]  SumI4OutMax=[]  SumDOutMin=[]  SumDOutMax=[]  DifferentiatorOutMin=[]  DifferentiatorOutMax=[]  FilterDiffOutCoefMin=[]  FilterDiffOutCoefMax=[]  ReciprocalOutMin=[]  ReciprocalOutMax=[]  SumDenOutMin=[]  SumDenOutMax=[]  SumNumOutMin=[]  SumNumOutMax=[]  DivideOutMin=[]  DivideOutMax=[]  UdiffTsProdOutMin=[]  UdiffTsProdOutMax=[]  NTsProdOutMin=[]  NTsProdOutMax=[]  UintegralTsProdOutMin=[]  UintegralTsProdOutMax=[]  UngainTsProdOutMin=[]  UngainTsProdOutMax=[]  ClampingZeroOutDataTypeStr=Inherit: Inherit via back propagation  ClampingZeroOutMin=[]  ClampingZeroOutMax=[]  FilterDenConstantOutDataTypeStr=Inherit: Inherit via back propagation  FilterDenConstantOutMin=[]  FilterDenConstantOutMax=[]  PCopyOutDataTypeStr=Inherit: Inherit via back propagation  PCopyOutMin=[]  PCopyOutMax=[]  NCopyOutDataTypeStr=Inherit: Inherit via back propagation  NCopyOutMin=[]  NCopyOutMax=[]  IntegratorContinuousStateAttributes=''  IntegratorStateMustResolveToSignalObject=off  IntegratorRTWStateStorageClass=Auto  FilterContinuousStateAttributes=''  FilterStateMustResolveToSignalObject=off  FilterRTWStateStorageClass=Auto  ParallelPVariant=InternalParameters  IdealPVariant=Disabled  IVariant=InternalParameters  DVariant=InternalParameters  IntegratorVariant=Continuous  SatVariant=Disabled  AWVariant=Passthrough  PCopyVariant=Disabled  TRVariant=Disabled  FdbkBlocksVariant=Forward  IdealPFdbkVariant=Disabled  SatFdbkVariant=Disabled  DerivativeFilterVariant=ContFilter  NVariant=InternalParameters  NCopyVariant=Disabled  FilterICVariant=InternalICsFilter  IntegratorICVariant=InternalICs  ExternalResetVariant=Disabled  TRSumVariant=Passthrough  SumFdbkVariant=Disabled  SumVariant=Sum_PID  TsampFilterVariant=InternalTs  TsampNgainVariant=Passthrough  TsampIntegralVariant=Disabled_SignalSpec  ExternalSaturationOutDataTypeStr=Inherit: Same as second input  DerivativeSourceVariant=ErrorSignal  PreIntVariant=InternalPreInt
  "roll pitch " : Scope  NumInputPorts=2
      settings: ActiveDisplayYMinimum=-0.54038754132904177  ActiveDisplayYMaximum=0.50630304776206048
  roll rate PID : slpidlib/PID Controller  Controller=PID  Form=Parallel  TimeDomain=Continuous-time  UseExternalTs=off  SampleTime=-1  IntegratorMethod=Forward Euler  FilterMethod=Forward Euler  ControllerParametersSource=internal  P=750  I=1500  UseKiTs=off  D=7.5  UseExternalDerivativeSource=off  N=100  UseFilter=on  TunerSelectOption=Transfer Function Based (PID Tuner App)  InitialConditionSource=internal  InitialConditionForIntegrator=0  InitialConditionForFilter=0  DifferentiatorICPrevScaledInput=0  ExternalReset=none  TrackingMode=off  Kt=1  LimitOutput=off  SatLimitsSource=internal  UpperSaturationLimit=inf  LowerSaturationLimit=-inf  LinearizeAsGain=on  AntiWindupMode=none  Kb=1  LimitIntegrator=off  UpperIntegratorSaturationLimit=inf  LowerIntegratorSaturationLimit=-inf  POutMin=[]  POutMax=[]  IOutMin=[]  IOutMax=[]  DOutMin=[]  DOutMax=[]  NOutMin=[]  NOutMax=[]  SumOutMin=[]  SumOutMax=[]  SaturationOutMin=[]  SaturationOutMax=[]  PParamMin=[]  PParamMax=[]  IParamMin=[]  IParamMax=[]  DParamMin=[]  DParamMax=[]  NParamMin=[]  NParamMax=[]  KbParamMin=[]  KbParamMax=[]  KtParamMin=[]  KtParamMax=[]  KbOutMin=[]  KbOutMax=[]  KtOutMin=[]  KtOutMax=[]  IntegratorOutMin=[]  IntegratorOutMax=[]  FilterOutMin=[]  FilterOutMax=[]  SumI1OutMin=[]  SumI1OutMax=[]  SumI2OutMin=[]  SumI2OutMax=[]  SumI3OutMin=[]  SumI3OutMax=[]  SumI4OutMin=[]  SumI4OutMax=[]  SumDOutMin=[]  SumDOutMax=[]  DifferentiatorOutMin=[]  DifferentiatorOutMax=[]  FilterDiffOutCoefMin=[]  FilterDiffOutCoefMax=[]  ReciprocalOutMin=[]  ReciprocalOutMax=[]  SumDenOutMin=[]  SumDenOutMax=[]  SumNumOutMin=[]  SumNumOutMax=[]  DivideOutMin=[]  DivideOutMax=[]  UdiffTsProdOutMin=[]  UdiffTsProdOutMax=[]  NTsProdOutMin=[]  NTsProdOutMax=[]  UintegralTsProdOutMin=[]  UintegralTsProdOutMax=[]  UngainTsProdOutMin=[]  UngainTsProdOutMax=[]  ClampingZeroOutDataTypeStr=Inherit: Inherit via back propagation  ClampingZeroOutMin=[]  ClampingZeroOutMax=[]  FilterDenConstantOutDataTypeStr=Inherit: Inherit via back propagation  FilterDenConstantOutMin=[]  FilterDenConstantOutMax=[]  PCopyOutDataTypeStr=Inherit: Inherit via back propagation  PCopyOutMin=[]  PCopyOutMax=[]  NCopyOutDataTypeStr=Inherit: Inherit via back propagation  NCopyOutMin=[]  NCopyOutMax=[]  IntegratorContinuousStateAttributes=''  IntegratorStateMustResolveToSignalObject=off  IntegratorRTWStateStorageClass=Auto  FilterContinuousStateAttributes=''  FilterStateMustResolveToSignalObject=off  FilterRTWStateStorageClass=Auto  ParallelPVariant=InternalParameters  IdealPVariant=Disabled  IVariant=InternalParameters  DVariant=InternalParameters  IntegratorVariant=Continuous  SatVariant=Disabled  AWVariant=Passthrough  PCopyVariant=Disabled  TRVariant=Disabled  FdbkBlocksVariant=Forward  IdealPFdbkVariant=Disabled  SatFdbkVariant=Disabled  DerivativeFilterVariant=ContFilter  NVariant=InternalParameters  NCopyVariant=Disabled  FilterICVariant=InternalICsFilter  IntegratorICVariant=InternalICs  ExternalResetVariant=Disabled  TRSumVariant=Passthrough  SumFdbkVariant=Disabled  SumVariant=Sum_PID  TsampFilterVariant=InternalTs  TsampNgainVariant=Passthrough  TsampIntegralVariant=Disabled_SignalSpec  ExternalSaturationOutDataTypeStr=Inherit: Same as second input  DerivativeSourceVariant=ErrorSignal  PreIntVariant=InternalPreInt
  "x and roll scope " : Scope  NumInputPorts=4
      settings: ActiveDisplayYMinimum=-4.2297316197274961  ActiveDisplayYMaximum=0.46997104179306176  DataLoggingVariableName=ScopeData3
  yaw : Scope  NumInputPorts=2
      settings: ActiveDisplayYMinimum=-0.313580624870494  ActiveDisplayYMaximum=1.0099890814182868  DataLoggingVariableName=ScopeData2
  yaw PID : slpidlib/PID Controller  Controller=PID  Form=Parallel  TimeDomain=Continuous-time  UseExternalTs=off  SampleTime=-1  IntegratorMethod=Forward Euler  FilterMethod=Forward Euler  ControllerParametersSource=internal  P=6  I=1  UseKiTs=off  D=0.35  UseExternalDerivativeSource=off  N=100  UseFilter=on  TunerSelectOption=Transfer Function Based (PID Tuner App)  InitialConditionSource=internal  InitialConditionForIntegrator=0  InitialConditionForFilter=0  DifferentiatorICPrevScaledInput=0  ExternalReset=none  TrackingMode=off  Kt=1  LimitOutput=off  SatLimitsSource=internal  UpperSaturationLimit=inf  LowerSaturationLimit=-inf  LinearizeAsGain=on  AntiWindupMode=none  Kb=1  LimitIntegrator=off  UpperIntegratorSaturationLimit=inf  LowerIntegratorSaturationLimit=-inf  POutMin=[]  POutMax=[]  IOutMin=[]  IOutMax=[]  DOutMin=[]  DOutMax=[]  NOutMin=[]  NOutMax=[]  SumOutMin=[]  SumOutMax=[]  SaturationOutMin=[]  SaturationOutMax=[]  PParamMin=[]  PParamMax=[]  IParamMin=[]  IParamMax=[]  DParamMin=[]  DParamMax=[]  NParamMin=[]  NParamMax=[]  KbParamMin=[]  KbParamMax=[]  KtParamMin=[]  KtParamMax=[]  KbOutMin=[]  KbOutMax=[]  KtOutMin=[]  KtOutMax=[]  IntegratorOutMin=[]  IntegratorOutMax=[]  FilterOutMin=[]  FilterOutMax=[]  SumI1OutMin=[]  SumI1OutMax=[]  SumI2OutMin=[]  SumI2OutMax=[]  SumI3OutMin=[]  SumI3OutMax=[]  SumI4OutMin=[]  SumI4OutMax=[]  SumDOutMin=[]  SumDOutMax=[]  DifferentiatorOutMin=[]  DifferentiatorOutMax=[]  FilterDiffOutCoefMin=[]  FilterDiffOutCoefMax=[]  ReciprocalOutMin=[]  ReciprocalOutMax=[]  SumDenOutMin=[]  SumDenOutMax=[]  SumNumOutMin=[]  SumNumOutMax=[]  DivideOutMin=[]  DivideOutMax=[]  UdiffTsProdOutMin=[]  UdiffTsProdOutMax=[]  NTsProdOutMin=[]  NTsProdOutMax=[]  UintegralTsProdOutMin=[]  UintegralTsProdOutMax=[]  UngainTsProdOutMin=[]  UngainTsProdOutMax=[]  ClampingZeroOutDataTypeStr=Inherit: Inherit via back propagation  ClampingZeroOutMin=[]  ClampingZeroOutMax=[]  FilterDenConstantOutDataTypeStr=Inherit: Inherit via back propagation  FilterDenConstantOutMin=[]  FilterDenConstantOutMax=[]  PCopyOutDataTypeStr=Inherit: Inherit via back propagation  PCopyOutMin=[]  PCopyOutMax=[]  NCopyOutDataTypeStr=Inherit: Inherit via back propagation  NCopyOutMin=[]  NCopyOutMax=[]  IntegratorContinuousStateAttributes=''  IntegratorStateMustResolveToSignalObject=off  IntegratorRTWStateStorageClass=Auto  FilterContinuousStateAttributes=''  FilterStateMustResolveToSignalObject=off  FilterRTWStateStorageClass=Auto  ParallelPVariant=InternalParameters  IdealPVariant=Disabled  IVariant=InternalParameters  DVariant=InternalParameters  IntegratorVariant=Continuous  SatVariant=Disabled  AWVariant=Passthrough  PCopyVariant=Disabled  TRVariant=Disabled  FdbkBlocksVariant=Forward  IdealPFdbkVariant=Disabled  SatFdbkVariant=Disabled  DerivativeFilterVariant=ContFilter  NVariant=InternalParameters  NCopyVariant=Disabled  FilterICVariant=InternalICsFilter  IntegratorICVariant=InternalICs  ExternalResetVariant=Disabled  TRSumVariant=Passthrough  SumFdbkVariant=Disabled  SumVariant=Sum_PID  TsampFilterVariant=InternalTs  TsampNgainVariant=Passthrough  TsampIntegralVariant=Disabled_SignalSpec  ExternalSaturationOutDataTypeStr=Inherit: Same as second input  DerivativeSourceVariant=ErrorSignal  PreIntVariant=InternalPreInt
  yaw rate PID : slpidlib/PID Controller  Controller=PID  Form=Parallel  TimeDomain=Continuous-time  UseExternalTs=off  SampleTime=-1  IntegratorMethod=Forward Euler  FilterMethod=Forward Euler  ControllerParametersSource=internal  P=360  I=16.7*3  UseKiTs=off  D=0  UseExternalDerivativeSource=off  N=100  UseFilter=on  TunerSelectOption=Transfer Function Based (PID Tuner App)  InitialConditionSource=internal  InitialConditionForIntegrator=0  InitialConditionForFilter=0  DifferentiatorICPrevScaledInput=0  ExternalReset=none  TrackingMode=off  Kt=1  LimitOutput=off  SatLimitsSource=internal  UpperSaturationLimit=inf  LowerSaturationLimit=-inf  LinearizeAsGain=on  AntiWindupMode=none  Kb=1  LimitIntegrator=off  UpperIntegratorSaturationLimit=inf  LowerIntegratorSaturationLimit=-inf  POutMin=[]  POutMax=[]  IOutMin=[]  IOutMax=[]  DOutMin=[]  DOutMax=[]  NOutMin=[]  NOutMax=[]  SumOutMin=[]  SumOutMax=[]  SaturationOutMin=[]  SaturationOutMax=[]  PParamMin=[]  PParamMax=[]  IParamMin=[]  IParamMax=[]  DParamMin=[]  DParamMax=[]  NParamMin=[]  NParamMax=[]  KbParamMin=[]  KbParamMax=[]  KtParamMin=[]  KtParamMax=[]  KbOutMin=[]  KbOutMax=[]  KtOutMin=[]  KtOutMax=[]  IntegratorOutMin=[]  IntegratorOutMax=[]  FilterOutMin=[]  FilterOutMax=[]  SumI1OutMin=[]  SumI1OutMax=[]  SumI2OutMin=[]  SumI2OutMax=[]  SumI3OutMin=[]  SumI3OutMax=[]  SumI4OutMin=[]  SumI4OutMax=[]  SumDOutMin=[]  SumDOutMax=[]  DifferentiatorOutMin=[]  DifferentiatorOutMax=[]  FilterDiffOutCoefMin=[]  FilterDiffOutCoefMax=[]  ReciprocalOutMin=[]  ReciprocalOutMax=[]  SumDenOutMin=[]  SumDenOutMax=[]  SumNumOutMin=[]  SumNumOutMax=[]  DivideOutMin=[]  DivideOutMax=[]  UdiffTsProdOutMin=[]  UdiffTsProdOutMax=[]  NTsProdOutMin=[]  NTsProdOutMax=[]  UintegralTsProdOutMin=[]  UintegralTsProdOutMax=[]  UngainTsProdOutMin=[]  UngainTsProdOutMax=[]  ClampingZeroOutDataTypeStr=Inherit: Inherit via back propagation  ClampingZeroOutMin=[]  ClampingZeroOutMax=[]  FilterDenConstantOutDataTypeStr=Inherit: Inherit via back propagation  FilterDenConstantOutMin=[]  FilterDenConstantOutMax=[]  PCopyOutDataTypeStr=Inherit: Inherit via back propagation  PCopyOutMin=[]  PCopyOutMax=[]  NCopyOutDataTypeStr=Inherit: Inherit via back propagation  NCopyOutMin=[]  NCopyOutMax=[]  IntegratorContinuousStateAttributes=''  IntegratorStateMustResolveToSignalObject=off  IntegratorRTWStateStorageClass=Auto  FilterContinuousStateAttributes=''  FilterStateMustResolveToSignalObject=off  FilterRTWStateStorageClass=Auto  ParallelPVariant=InternalParameters  IdealPVariant=Disabled  IVariant=InternalParameters  DVariant=InternalParameters  IntegratorVariant=Continuous  SatVariant=Disabled  AWVariant=Passthrough  PCopyVariant=Disabled  TRVariant=Disabled  FdbkBlocksVariant=Forward  IdealPFdbkVariant=Disabled  SatFdbkVariant=Disabled  DerivativeFilterVariant=ContFilter  NVariant=InternalParameters  NCopyVariant=Disabled  FilterICVariant=InternalICsFilter  IntegratorICVariant=InternalICs  ExternalResetVariant=Disabled  TRSumVariant=Passthrough  SumFdbkVariant=Disabled  SumVariant=Sum_PID  TsampFilterVariant=InternalTs  TsampNgainVariant=Passthrough  TsampIntegralVariant=Disabled_SignalSpec  ExternalSaturationOutDataTypeStr=Inherit: Same as second input  DerivativeSourceVariant=ErrorSignal  PreIntVariant=InternalPreInt
  Rotor 1 PWM : Outport
  Rotor 2 PWM : Outport  Port=2
  Rotor 3 PWM : Outport  Port=3
  Rotor 4 PWM : Outport  Port=4
  wires:
  hover_voltage keep?/1 -> Sum4/1, Sum7/1, Sum6/1, Sum5/1
  Sum13/1 -> Rotor 3 PWM/1, PWM scope/3  "voltage 3"
  Sum11/1 -> Rotor 1 PWM/1, PWM scope/1  "voltage 1"
  Sum4/1 -> Sum9/3
  Sum6/1 -> Sum14/3
  opposite spin4/1 -> Rotor 4 PWM/1, PWM scope/4  "voltage 4"
  opposite spin2/1 -> Rotor 2 PWM/1, PWM scope/2  "voltage 2"
  ref z/1 -> Sum/1, Scope/1
  z/1 -> Sum/2, Scope/2
  Sum/1 -> height PID/1  "z_error"
  x/1 -> Sum2/2
  Sum2/1 -> "x and roll scope "/1  "x_error"
  ref roll/1 -> Mux/1, Sum10/1
  roll_y/1 -> Mux/2, Sum10/2
  Sum10/1 -> roll PID/1, "x and roll scope "/2  "roll_error"
  max roll pwm/1 -> Sum11/4, Sum14/4, Sum13/4, Sum9/4, Roll Pitch Yaw PWM/1, "x and roll scope "/3  "roll voltage"
  roll PID/1 -> Sum12/1  "droll ref"
  droll/1 -> Sum12/2
  Sum12/1 -> roll rate PID/1
  roll rate PID/1 -> max roll pwm/1, "x and roll scope "/4
  Sum8/1 -> pitch rate PID/1
  dpitch/1 -> Sum8/2
  pitch PID/1 -> Sum8/1  "dpitch ref"
  Sum3/1 -> pitch PID/1  "pitch_error"
  pitch_x/1 -> Mux1/2, Sum3/2
  ref pitch/1 -> Mux1/1, Sum3/1
  Sum5/1 -> Sum13/3
  Sum14/1 -> opposite spin2/1
  Sum9/1 -> opposite spin4/1
  Sum7/1 -> Sum11/3
  pitch rate PID/1 -> max pitch pwm/1
  max pitch pwm/1 -> Sum11/1, Sum14/1, Sum13/1, Sum9/1, Roll Pitch Yaw PWM/2  "pitch voltage"
  yaw rate PID/1 -> max yaw pwm/1
  ref yaw/1 -> yaw/1, Sum15/1
  yaw_z/1 -> yaw/2, Sum15/2
  Sum15/1 -> yaw PID/1  "yaw_error"
  yaw PID/1 -> Sum16/1  "dyaw ref"
  dyaw/1 -> Sum16/2
  Sum16/1 -> yaw rate PID/1
  max yaw pwm/1 -> Sum11/2, Sum14/2, Sum13/2, Sum9/2, Roll Pitch Yaw PWM/3  "yaw voltage"
  height PID/1 -> Sum7/2, Sum5/2, Sum6/2, Sum4/2
  Mux/1 -> "roll pitch "/1
  Mux1/1 -> "roll pitch "/2
